simulink model "Porsche930Turbo_Model_V0"  (R2025b)
settings: Solver=ode3  StartTime=0.0  StopTime=1800  FixedStep=0.005  MaxStep=0.01  RelTol=1e-3
values from neighbouring files (symbols this model uses):
  a_front = (1 - CoG_front) * wb    (= 1.32912)    [Main.m]
  af = 1.77    [Main.m]
  bsfc = 395    [Main.m]
  cd = 0.39    [Main.m]
  crr = 0.015    [Main.m]
  distance_imola = s_track    [Main.m]
  eta_gb = 0.95    [Main.m]
  gear_numbers = [1, 2, 3, 4]    [Main.m]
  gear_ratios = [2.25, 1.30, 0.89, 0.625]    [Main.m]
  gear_shift_tbl = [1, 2, 3, 4]    [Main.m]
  grade_imola = grade_track    [Main.m]
  kt = 1.65    [Main.m]
  m_eq = mg + (J_wheels / rw^2) + (J_drivetrain * i_avg^2 / rw^2)    [Main.m]
  mg = mc + (mh * np) + mp_hybrid    (= 1492.5)    [Main.m]
  mu_road = 0.9    [Main.m]
  n_ice = 0:dn:nd    [Main.m]
  ne_em = 0:dn:nemax_em    [Main.m]
  nparallel = 2    [Main.m]
  nseries = 96    [Main.m]
  rho_fuel = 0.75    [Main.m]
  ro = 1.204    [Main.m]
  rt = 4.222    [Main.m]
  rw = (dw * 25.4 / 2 + wt * art / 100) * 1e-3    (= 0.31345)    [Main.m]
  t_ice = zeros(size(n_ice))    [Main.m]
  t_roma_san_basilio = [0 1 2 3 4 5 6 7 8 9 10 11 ... (522 elements, 522x1)]    [ECE_EUDC_Artemis_Bologna_Roma_WLTC_EE_bus.mat]
  tau_turbo = 0.6    [Main.m]
  te_em = zeros(size(ne_em))    [Main.m]
  te_em_peak = zeros(size(ne_em))    [Main.m]
  temax_em = 230    [Main.m]
  tmax_ice = 412    [Main.m]
  track_length = 4909    [Main.m]
  v_cutoff_bp = [0, 0.5, 1.4, 50]    [Main.m]
  v_cutoff_tbl = [0, 0,   1,   1 ]    [Main.m]
  v_ref_imola = v_track_ms    [Main.m]
  v_shift_bp = [0, 18, 33, 48]    [Main.m]
  v_shift_bp_EMODE = [0, 5, 22, 35]    [Main.m]
  vkm_roma_san_basilio = [28.8 30.9 32.4 34.2 35.3 35.6 34.8 33.8 32.2 30.5 29.1 27.9 ... (522 elements, 522x1)]    [ECE_EUDC_Artemis_Bologna_Roma_WLTC_EE_bus.mat]
  wb = 2.272    [Main.m]
undefined symbols (not defined in the file or in its folder): SoC_Per
libraries: simulink x58
(part 1 of 5)
settings Model: Creator=testi  LastModifiedBy=emanu
settings SolverCC: ConsecutiveZCsStepRelTol=1e-5  ZeroCrossAlgorithm=Adaptive
settings DebuggingCC: MergeDetectMultiDrivingBlocksExec=none  MaxConsecutiveZCsMsg=none  IgnoredZcDiagnostic=none
settings ModelReferenceCC: PropagateSignalLabelsOutOfModel=off

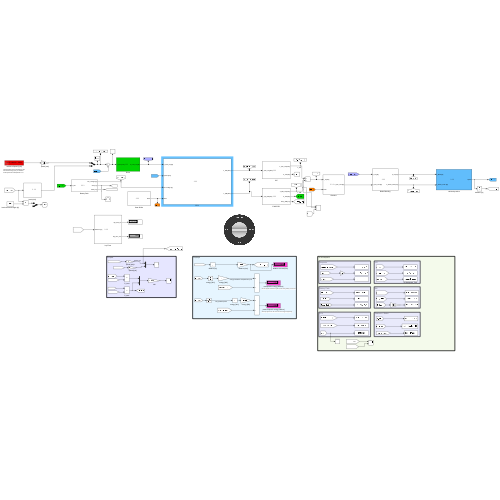
[thumbnail: Simulink's stored preview of the top-level diagram]
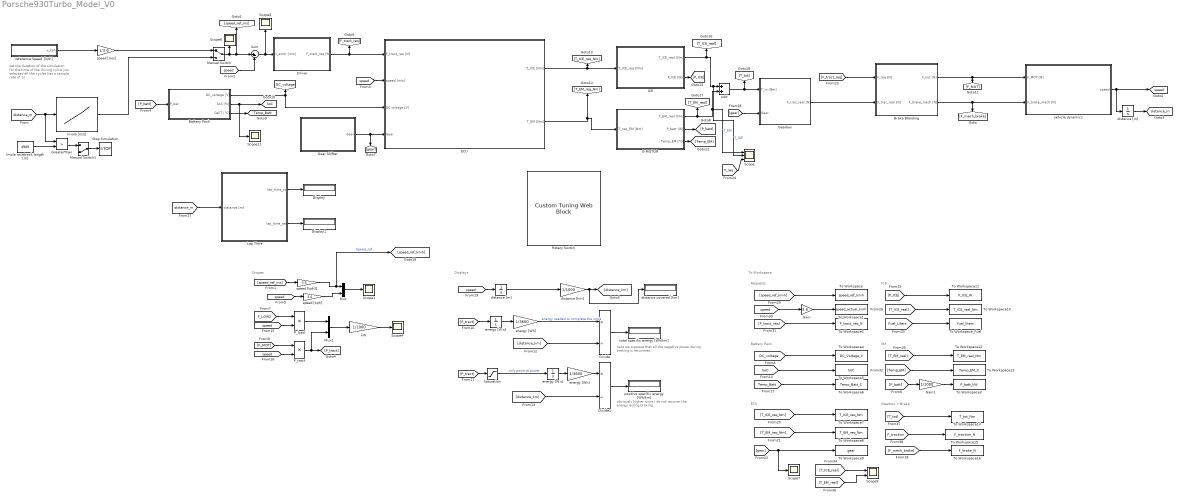
== system Porsche930Turbo_Model_V0 ==
  note: Gearbox + Brake
  note: EM
  note: ICE
  note: ECU
  note: Requests
  note: To Workspace
  note: set the duration of the simulation for the time of the driving cylce you selected
      | all the cycles has a sample rate of 1s
  note: Displays
  note: Scopes
  note: here we suppose that all the negative power during braking is recovered
  note: obviously higher since I do not recover the energy during braking
  note: Battery Pack
  Add : Sum
  Battery Pack : Subsystem
      mask Display: image('battery.jpg');
  Brake Blending : Subsystem
      mask Display: image('drumbrake.jpg');
  Display : Display
  Display1 : Display
  Divide : Product  Inputs=*/
  Divide1 : Product  Inputs=*/
  Driver : Subsystem
      mask Display: image('driver.webp');
  E-MOTOR : Subsystem
      mask Display: image('EMOTOR.jpg');
  ECU : Subsystem
      mask Display: image('ECU.webp');
  Gain : Gain  Gain=3.6
  Gain1 : Gain  Gain=1/1000
  Gear Shifter : Subsystem
      mask Display: image('Gearstick.jpeg');
  Gearbox : Subsystem
      mask Display: image('Gearbox.jpg');
  GreaterThan : RelationalOperator  Operator=>  OutDataTypeStr=boolean  RndMeth=Simplest  InputSameDT=off
  ICE : Subsystem
      mask Display: image('ICE.jpg');
  Imola [m/s] : Lookup_n-D  NumberOfTableDimensions=1  BreakpointsForDimension1=distance_imola  Table=v_ref_imola  InternalRulePriority=Speed  RndMeth=Simplest
      mask Display: image('imola.webp');
  Imola racetrack length [m] : Constant  Value=4909
  Lap TIme : Subsystem
      mask Display: image('clock.webp');
  Manual Switch : ManualSwitch
  Manual Switch1 : ManualSwitch  CurrentSetting=0
  Mux : Mux  Inputs=2
  Mux2 : Mux  Inputs=2
  P_load : Product
  P_tract : Product
  Rotary Switch : CustomTuningWebBlock  LabelPosition=Hide  ShowInitialText=on  Configuration="{\"components\":[{\"name\":\"RotarySwitchComponent\",\"settings\":{\"arcAngle\":270,\"arcAngleOffset\":180,\"handle\":{\"size\":[150,150],\"src\":\"data:image\\/svg+xml;base64,PHN2ZyBpZD0iTGF5ZXJfMSIgZGF0YS1uYW1lPSJMYXllciAxIiB4bWxucz0iaHR0cDovL3d3dy53My5vcmcvMjAwMC9zdmciIHhtbG5zOnhsaW5rPSJodHRwOi8vd3d3LnczLm9yZy8xOTk5L3hsaW5rIiB2aWV3Qm94PSIwIDAgMTIxIDEyMSI+PGRlZnM+PHN0eWxlPi5jbHMtMXtmaWxsOnVybCgjbGluZWFyLWdyYWRpZW50KTt9LmNscy0yLC5jbHMtM3tmaWxsOiNkMWQxZDE7fS5jbHMtM3tzdHJva2U6I2I3YjdiNztzdHJva2UtbWl0ZXJsaW1pdDoxMDtzdHJva2Utd2lkdGg6MC4yNXB4O30uY2xzLTR7ZmlsbDojZjMwMDAwO30uY2xzLTV7ZmlsbDojZjIxNzY3O308L3N0eWxlPjxsaW5lYXJHcmFkaWVudCBpZD0ibGluZWFyLWdyYWRpZW50IiB4MT0iNjAuNSIgeTE9IjEyMC41IiB4Mj0iNjAuNSIgeTI9IjAuNSIgZ3JhZGllbnRVbml0cz0idXNlclNwYWNlT25Vc2UiPjxzdG9wIG9mZnNldD0iMCIgc3RvcC1jb2xvcj0iI2QxZDFkMSIvPjxzdG9wIG9mZnNldD0iMC4xIiBzdG9wLWNvbG9yPSIjY2VjZWNlIi8+PHN0b3Agb2Zmc2V0PSIwLjE5IiBzdG9wLWNvbG9yPSIjYzNjM2MzIi8+PHN0b3Agb2Zmc2V0PSIwLjI4IiBzdG9wLWNvbG9yPSIjYjFiMWIxIi8+PHN0b3Agb2Zmc2V0PSIwLjM2IiBzdG9wLWNvbG9yPSIjOTg5ODk4Ii8+PHN0b3Agb2Zmc2V0PSIwLjQ0IiBzdG9wLWNvbG9yPSIjNzg3ODc4Ii8+PHN0b3Agb2Zmc2V0PSIwLjQ2IiBzdG9wLWNvbG9yPSIjNmI2YjZiIi8+PHN0b3Agb2Zmc2V0PSIwLjU0IiBzdG9wLWNvbG9yPSIjNmI2YjZiIi8+PHN0b3Agb2Zmc2V0PSIwLjU2IiBzdG9wLWNvbG9yPSIjNzY3Njc2Ii8+PHN0b3Agb2Zmc2V0PSIwLjY0IiBzdG9wLWNvbG9yPSIjOTc5Nzk3Ii8+PHN0b3Agb2Zmc2V0PSIwLjcyIiBzdG9wLWNvbG9yPSIjYjBiMGIwIi8+PHN0b3Agb2Zmc2V0PSIwLjgxIiBzdG9wLWNvbG9yPSIjYzNjM2MzIi8+PHN0b3Agb2Zmc2V0PSIwLjkiIHN0b3AtY29sb3I9IiNjZGNkY2QiLz48c3RvcCBvZmZzZXQ9IjEiIHN0b3AtY29sb3I9IiNkMWQxZDEiLz48L2xpbmVhckdyYWRpZW50PjwvZGVmcz48Y2lyY2xlIGNsYXNzPSJjbHMtMSIgY3g9IjYwLjUiIGN5PSI2MC41IiByPSI2MCIvPjxwYXRoIGNsYXNzPSJjbHMtMiIgZD0iTTYwLjUsMUE1OS41LDU5LjUsMCwxLDEsMSw2MC41LDU5LjU3LDU5LjU3LDAsMCwxLDYwLjUsMW0wLTFBNjAuNSw2MC41LDAsMSwwLDEyMSw2MC41LDYwLjUsNjAuNSwwLDAsMCw2MC41LDBaIi8+PHJlY3QgY2xhc3M9ImNscy0zIiB4PSIwLjUiIHk9IjUxLjUiIHdpZHRoPSIxMjAiIGhlaWdodD0iMTgiIHJ4PSIzLjA0Ii8+PHJlY3QgY2xhc3M9ImNscy00IiB4PSI1Ljc1IiB5PSI1OC43NSIgd2lkdGg9IjE2IiBoZWlnaHQ9IjMiLz48cGF0aCBjbGFzcz0iY2xzLTUiIGQ9Ik0yMS4yNSw1OS4yNXYyaC0xNXYtMmgxNW0xLTFoLTE3djRoMTd2LTRaIi8+PC9zdmc+\"},\"handleOffset\":[0,0],\"handleOrientation\":180,\"handlePosition\":[0,0,1,1],\"handleSize\":{\"height\":0.5,\"width\":0.5},\"labelRadius\":0.4,\"position\":[0,0,1,1],\"states\":[{\"Label\":{\"color\":[0,0,0,1],\"icon\":{\"size\":[0,0],\"src\":[],\"srcOrientation\":\"Right\"},\"iconOffset\":0,\"iconPlacement\":\"left\",\"opacity\":1,\"position\":[0.7345552884615385,0.6796274038461538],\"show\":true,\"text\":{\"content\":\"ICE\",\"font\":\"Helvetica\"}},\"Value\":1},{\"Label\":{\"color\":[0,0,0,1],\"icon\":{\"size\":[0,0],\"src\":[],\"srcOrientation\":\"Right\"},\"iconOffset\":0,\"iconPlacement\":\"left\",\"opacity\":1,\"position\":[0.35757211538461536,0.7603966346153846],\"show\":true,\"text\":{\"content\":\"ELECTRIC\",\"font\":\"Helvetica\"}},\"Value\":2},{\"Label\":{\"color\":[0,0,0,1],\"icon\":{\"size\":[0,0],\"src\":[],\"srcOrientation\":\"Right\"},\"iconOffset\":0,\"iconPlacement\":\"left\",\"opacity\":1,\"position\":[0.09603365384615385,0.46033653846153844],\"show\":true,\"text\":{\"content\":\"HYBRID\",\"font\":\"Helvetica\"}},\"Value\":3},{\"Label\":{\"color\":[0,0,0,1],\"icon\":{\"size\":[0,0],\"src\":[],\"srcOrientation\":\"Right\"},\"iconOffset\":0,\"iconPlacement\":\"left\",\"opacity\":1,\"position\":[0.36532451923076925,0.1180889423076923],\"show\":true,\"text\":{\"content\":\"RACE\",\"font\":\"Helvetica\"}},\"Value\":4}],\"tickRadius\":0.32}},{\"name\":\"BackgroundImageComponent\",\"settings\":{\"image\":{\"size\":[155,150],\"src\":\"data:image\\/svg+xml;base64,PD94bWwgdmVyc2lvbj0iMS4wIiBlbmNvZGluZz0idXRmLTgiPz4NCjwhLS0gR2VuZXJhdG9yOiBBZG9iZSBJbGx1c3RyYXRvciAyNS4wLjAsIFNWRyBFeHBvcnQgUGx1Zy1JbiAuIFNWRyBWZXJzaW9uOiA2LjAwIEJ1aWxkIDApICAtLT4NCjxzdmcgdmVyc2lvbj0iMS4xIg0KCSBpZD0iTGF5ZXJfMl8xXyIgeG1sbnM6Y2M9Imh0dHA6Ly9jcmVhdGl2ZWNvbW1vbnMub3JnL25zIyIgeG1sbnM6ZGM9Imh0dHA6Ly9wdXJsLm9yZy9kYy9lbGVtZW50cy8xLjEvIiB4bWxuczppbmtzY2FwZT0iaHR0cDovL3d3dy5pbmtzY2FwZS5vcmcv ...(+4184 chars)\",\"srcOrientation\":\"Right\"},\"position\":[0,0,1,1],\"scaleMode\":\"0\"}},{\"name\":\"ForegroundImageComponent\",\"settings\":{\"image\":{\"size\":[0,0],\"src\":\"default\",\"srcOrientation\":[]},\"isForeground\":1,\"position\":[0,0,1,1],\"scaleMode\":\"0\"}}],\"derived\":{\"blockParameters\":{\"ForegroundColor\":[0.9176470588235294,0.9176470588235294,0.9176470588235294],\"SelectedStateIndex\":0,\"States\":[{\"Label\":{\"color\":[0,0,0,1],\"icon\":{\"size\":[0,0],\"src\":[],\"srcOrientation\":\"Right\"},\"iconOffset\":0,\"iconPlacement\":\"left\",\"opacity\":1,\"position\":[0.7345552884615385,0.6796274038461538],\"show\":true,\"text\":{\"content\":\"ICE\",\"font\":\"Helvetica\"}},\"Value\":1},{\"Label\":{\"color\":[0,0,0,1],\"icon\":{\"size\":[0,0],\"src\":[],\"srcOrientation\":\"Right\"},\"iconOffset\":0,\"iconPlacement\":\"left\",\"opacity\":1,\"position\":[0.35757211538461536,0.7603966346153846],\"show\":true,\"text\":{\"content\":\"ELECTRIC\",\"font\":\"Helvetica\"}},\"Value\":2},{\"Label\":{\"color\":[0,0,0,1],\"icon\":{\"size\":[0,0],\"src\":[],\"srcOrientation\":\"Right\"},\"iconOffset\":0,\"iconPlacement\":\"left\",\"opacity\":1,\"position\":[0.09603365384615385,0.46033653846153844],\"show\":true,\"text\":{\"content\":\"HYBRID\",\"font\":\"Helvetica\"}},\"Value\":3},{\"Label\":{\"color\":[0,0,0,1],\"icon\":{\"size\":[0,0],\"src\":[],\"srcOrientation\":\"Right\"},\"iconOffset\":0,\"iconPlacement\":\"left\",\"opacity\":1,\"position\":[0.36532451923076925,0.1180889423076923],\"show\":true,\"text\":{\"content\":\"RACE\",\"font\":\"Helvetica\"}},\"Value\":4}],\"StatesJSON\":[{\"Label\":\"ICE\",\"Value\":1},{\"Label\":\"ELECTRIC\",\"Value\":2},{\"Label\":\"HYBRID\",\"Value\":3},{\"Label\":\"RACE\",\"Value\":4}],\"enumDataType\":\"\",\"fixedAspectRatio\":\"on\",\"useEnumDataType\":false}},\"settings\":{\"BindingType\":\"param\",\"backgroundColor\":[0,0,255,\"1\"],\"backgroundOffset\":1,\"fixedAspectRatio\":\"on\",\"image\":{\"size\":[150,150],\"src\":\"data:image\\/svg+xml;base64,PD94bWwgdmVyc2lvbj0iMS4wIiBlbmNvZGluZz0iVVRGLTgiIHN0YW5kYWxvbmU9Im5vIj8+CjwhLS0gR2VuZXJhdG9yOiBBZG9iZSBJbGx1c3RyYXRvciAxOS4yLjEsIFNWRyBFeHBvcnQgUGx1Zy1JbiAuIFNWRyBWZXJzaW9uOiA2LjAwIEJ1aWxkIDApICAtLT4KCjxzdmcKICAgeG1sbnM6ZGM9Imh0dHA6Ly9wdXJsLm9yZy9kYy9lbGVtZW50cy8xLjEvIgogICB4bWxuczpjYz0iaHR0cDovL2NyZWF0aXZlY29tbW9ucy5vcmcvbnMjIgogICB4bWxuczpyZGY9Imh0dHA6Ly93d3cudzMub3JnLzE5OTkvMDIvMjItcmRmLXN5bnRh ...(+9660 chars)\"},\"showBackgroundColor\":false,\"variant\":\"rotarySwitch\",\"version\":\"R2023a\"},\"type\":\"RotarySwitch\"}"  CustomBackgroundColor="{\"color\":[0,0,0],\"show\":true}"
  Saturation : Saturate  UpperLimit=inf  LowerLimit=0
  Scope : Scope  NumInputPorts=3
      settings: ActiveDisplayYMinimum=-46.9478660870644  ActiveDisplayYMaximum=422.53079478357967  DataLoggingVariableName=ScopeData11
  Scope{1,4..7,11} (6 alike) : Scope
      Scope1 settings: ActiveDisplayYMinimum=-21.249999999999996  ActiveDisplayYMaximum=191.25  DataLoggingVariableName=ScopeData18
      Scope11 settings: ActiveDisplayYMinimum=0.17583888024091721  ActiveDisplayYMaximum=0.417415089905262  DataLoggingVariableName=ScopeData37
      Scope4 settings: DataLoggingVariableName=ScopeData23
      Scope5 settings: ActiveDisplayYMinimum=-1  ActiveDisplayYMaximum=1  DataLoggingVariableName=ScopeData21
      Scope6 settings: ActiveDisplayYMinimum=-2.2361111111111112  ActiveDisplayYMaximum=20.125000000000004  DataLoggingVariableName=ScopeData22
      Scope7 settings: ActiveDisplayYMinimum=-1  ActiveDisplayYMaximum=1  DataLoggingVariableName=ScopeData29
  Scope9 : Scope  NumInputPorts=2
      settings: ActiveDisplayYMinimum=-51.4997582842605  ActiveDisplayYMaximum=463.49782455834463  DataLoggingVariableName=ScopeData31
  Stop Simulation : Stop
  Sum : Sum  Inputs=|+-
  To Workspace : ToWorkspace  VariableName=speed_ref_kmh  SampleTime=-1
  To Workspace1 : ToWorkspace  VariableName=speed_actual_kmh  SampleTime=-1
  To Workspace10 : ToWorkspace  VariableName=T_ICE_real_Nm  SampleTime=-1
  To Workspace11 : ToWorkspace  VariableName=P_ICE_W  SampleTime=-1
  To Workspace12 : ToWorkspace  VariableName=T_EM_real_Nm  SampleTime=-1
  To Workspace13 : ToWorkspace  VariableName=Temp_EM_C  SampleTime=-1
  To Workspace14 : ToWorkspace  VariableName=T_tot_Nm  SampleTime=-1
  To Workspace15 : ToWorkspace  VariableName=F_traction_N  SampleTime=-1
  To Workspace16 : ToWorkspace  VariableName=F_brake_N  SampleTime=-1
  To Workspace2 : ToWorkspace  VariableName=F_tract_req_N  SampleTime=-1
  To Workspace3 : ToWorkspace  VariableName=P_batt_kW  SampleTime=-1
  To Workspace4 : ToWorkspace  VariableName=DC_Voltage_V  SampleTime=-1
  To Workspace5 : ToWorkspace  VariableName=SoC  SampleTime=-1
  To Workspace6 : ToWorkspace  VariableName=Temp_Batt_C  SampleTime=-1
  To Workspace7 : ToWorkspace  VariableName=T_ICE_req_Nm  SampleTime=-1
  To Workspace8 : ToWorkspace  VariableName=T_EM_req_Nm  SampleTime=-1
  To Workspace9 : ToWorkspace  VariableName=gear  SampleTime=-1
  To Workspace_Fuel : ToWorkspace  VariableName=fuel_liters  SampleTime=-1
  distance [km] : Gain  Gain=1/1000
  distance [m] : Integrator
  "distance [m] " : Integrator
  distance covered [km] : Display
  energy [W.s] : Integrator
  "energy [W.s] " : Integrator
  energy [Wh] : Gain  Gain=1/3600
  "energy [Wh] " : Gain  Gain=1/3600
  kW : Gain  Gain=1/1000
  positive specific energy [Wh/km] : Display
  reference Speed  [kph] : Subsystem  mask{slct=WLTC class3b - 1800s}
      mask prompts: slct "Select Cycle"
      mask help: by mtb
      mask init:
      | load('ECE_EUDC_Artemis_Bologna_Roma_WLTC_EE_bus.mat')
      mask TypeOptions slct: ECE15 - 195s | EUDC - 400s | Art. Urban - 994s | Art. Rural - 1083s | Art. Motorway - 1068s | Roma S.Basilio - 522s | BO Viali slow - 1321s | BO Viali quick - 1215s | WLTC city - 1022s | WLTC class1 - 1612s | WLTC class2 - 1800s | WLTC class3a - 1800s | WLTC class3b - 1800s | Bus line BO 27A - 3246s | Bus line BO 27B - 3058s | Bus line BO 33 - 1850s | EE Bike Cycle - 1201s | 130kph
      mask DialogControl DescGroupVar Prompt: LEMAD Speed Cycle
      mask DialogControl DescTextVar Prompt: Function that outputs the speed reference in Km/h for the desired cycle
      mask Display:
      | switch slct
      |     case 1
      |         fprintf('ECE15 - 195s');
      |     case 2
      |         fprintf('EUDC - 400s');
      |     case 3
      |         fprintf('Art. Urban - 994s');
      |     case 4
      |         fprintf('Art. Rural - 1083s');
      |     case 5
      |         fprintf('Art. Motorway - 1068s');
      |     case 6
      |         fprintf('Roma S.Basilio - 522s');
      |     case 7
      |         fprintf('BO Viali slow - 1321s');
      |     case 8
      |         fprintf('BO Viali quick - 1215s');
      |     case 9
      |         fprintf('WLTC city - 1022s');
      |     case 10
      |         fprintf('WLTC class1 - 1612s');
      |     case 11
      |         fprintf('WLTC class2 - 1800s');
      |     case 12
      |         fprintf('WLTC class3a - 1800s');
      |     case 13
      |         fprintf('WLTC class3b - 1800s');
      |     case 14
      |         fprintf('Bus line BO 27A - 3246s');
      |     case 15
      |         fprintf('Bus line BO 27A - 3058s');
      |     case 16
      |         fprintf('Bus line BO 33 - 1850s');
      |     case 17
      |         fprintf('EE Bike Cycle - 1201s');
      |     case 18
      |         fprintf('130kph');
      | end
  speed [kph] : Gain  Gain=3.6
  speed [kph]1 : Gain  Gain=3.6
  speed [m/s] : Gain  Gain=1/3.6
  total specific energy [Wh/km] : Display
  vehicle dynamics : Subsystem
      mask Display: image('930_turbo_050.webp');
  tag scope: DC_voltage=global, SoC=global, Temp_Batt=global, distance_m=global, speed=global
  wires:
  Sum/1 -> Driver/1(v_error [m/s]), Scope5/1
  Driver/1(F_tract_req [N]) -> [F_tract_req], ECU/1(F_tract_req [N])
  Battery Pack/1(DC_voltage [V]) -> ECU/3(DC voltage [V]), [DC_voltage]
  ECU/1(T_ICE [Nm]) -> ICE/1(T_ICE_req [Nm]), [T_ICE_req_Nm]
  ICE/1(T_ICE_real [Nm]) -> [T_ICE_real], Scope/2, Add/1  "T_ICE"
  [P_tract] -> energy [W.s]/1
  Mux2/1 -> kW/1
  [distance_km] -> Divide1/2
  Saturation/1 -> "energy [W.s] "/1  "only positive power"
  "energy [Wh] "/1 -> Divide1/1
  kW/1 -> Scope4/1
  Divide1/1 -> positive specific energy [Wh/km]/1
  P_tract/1 -> Mux2/2, [P_tract]
  "energy [W.s] "/1 -> "energy [Wh] "/1
  [speed] -> speed [kph]/1
  Mux/1 -> Scope1/1
  [F_LOAD] -> P_load/1
  [speed] -> P_tract/2
  energy [Wh]/1 -> Divide/1  "energy needed to complete the cycle"
  [distance_km] -> Divide/2
  [P_tract] -> Saturation/1
  [speed] -> distance [m]/1
  [speed] -> P_load/2
  [speed_ref_ms] -> speed [kph]1/1
  distance [km]/1 -> distance covered [km]/1, [distance_km]
  speed [kph]/1 -> Mux/2
  Divide/1 -> total specific energy [Wh/km]/1
  [F_MOT] -> P_tract/1
  energy [W.s]/1 -> energy [Wh]/1
  P_load/1 -> Mux2/1
  distance [m]/1 -> distance [km]/1
  [F_tract_req] -> Brake Blending/1(F_req [N])
  Brake Blending/1(F_out [N]) -> [F_MOT], vehicle dynamics/1(F_MOT [N])
  Brake Blending/2(F_brake_mech [N]) -> vehicle dynamics/2(F_brake_mech [N]), [F_mech_brake]
  [P_batt] -> Battery Pack/1(P_bat)
  vehicle dynamics/1(speed) -> "distance [m] "/1, [speed]
  "distance [m] "/1 -> [distance_m]
  [distance_m] -> GreaterThan/1, Imola [m/s]/1
  Imola [m/s]/1 -> Manual Switch/2
  speed [m/s]/1 -> Manual Switch/1
  Manual Switch/1 -> [speed_ref_ms], Sum/1, Scope6/1
  Add/1 -> [T_tot], Gearbox/1(T_in [Nm])
  Imola racetrack length [m]/1 -> GreaterThan/2
  [gear] -> Gearbox/2(Gear)
  Gearbox/1(F_trac_real [N]) -> Brake Blending/2(F_trac_real [N])
  E-MOTOR/2(P_batt [W]) -> [P_batt]
  Battery Pack/3(CellT [°C]) -> [Temp_Batt]
  E-MOTOR/1(T_EM_real [Nm]) -> [T_EM_real], Add/2, Scope/1  "T_EM"
  Battery Pack/2(SoC [%]) -> Scope11/1, [SoC]
  [distance_m] -> Lap TIme/1(distance [m])
  Lap TIme/1(lap_time_str) -> Display/1
  Lap TIme/2(lap_time_sec) -> Display1/1
  reference Speed  [kph]/1(v_kph) -> speed [m/s]/1
  GreaterThan/1 -> Manual Switch1/1
  Manual Switch1/1 -> Stop Simulation/1
  E-MOTOR/3(Temp_EM [°C]) -> [Temp_EM]
  [speed] -> Gain/1
  [speed_ref_kmh] -> To Workspace/1
  Gain/1 -> To Workspace1/1
  [F_tract_req] -> To Workspace2/1
  [SoC] -> To Workspace5/1
  [DC_voltage] -> To Workspace4/1
  [Temp_Batt] -> To Workspace6/1
  [speed] -> ECU/2(speed [m/s])
  [speed] -> Sum/2
  ECU/2(T_EM [Nm]) -> [T_EM_req_Nm], E-MOTOR/1(T_req_EM [Nm])
  [T_ICE_req_Nm] -> To Workspace7/1
  [T_EM_req_Nm] -> To Workspace8/1
  [gear] -> Scope7/1, To Workspace9/1
  ICE/2(P_ICE [W]) -> [P_ICE]
  [Fuel_Liters] -> To Workspace_Fuel/1
  [T_ICE_real] -> To Workspace10/1
  [P_ICE] -> To Workspace11/1
  [T_ICE_real] -> Scope9/1
  [P_batt] -> Gain1/1
  Gain1/1 -> To Workspace3/1
  [Temp_EM] -> To Workspace13/1
  [T_EM_real] -> To Workspace12/1
  [T_EM_real] -> Scope9/2
  [T_tot] -> To Workspace14/1
  [F_traction] -> To Workspace15/1
  Gear Shifter/1(Gear) -> ECU/4(Gear), [gear]
  [F_mech_brake] -> To Workspace16/1
  speed [kph]1/1 -> [speed_ref_kmh], Mux/1  "Speed_ref"
  [T_req] -> Scope/3

== system Porsche930Turbo_Model_V0/Battery Pack ==
  P_bat : Inport
  " " : Product  Inputs=*/
  Constant : Constant  Value=25
  Constant1 : Constant  Value=nparallel
  Constant2 : Constant  Value=nseries
  Data Type Conversion : DataTypeConversion  SaturateOnIntegerOverflow=off  RndMeth=Floor
  Gain2 : Gain  Gain=1/100
  Memory : Memory  InitialCondition=345.2
  P_tract1 : Product  Inputs=3
  Scope : Scope
      settings: ActiveDisplayYMinimum=271.806844329834  ActiveDisplayYMaximum=353.35479507446286  DataLoggingVariableName=ScopeData36
  Scope2 : Scope  NumInputPorts=4
      settings: Title=BATTERY VOLTAGE  ActiveDisplayYMinimum=338.44709014892578  ActiveDisplayYMaximum=434.32286834716797  DataLoggingSaveFormat=Array
  Subsystem : Subsystem  mask{seriesNumber=96, parallelNumber=2, InitialSOC=SoC_Per, InitialSOH=100.0, BattEff=98.0, CellType=MOLICEL	21700	P42A	4.2 [Ah], ThermalModelType=1D With Plastic, ThermReff=off, TRoom=20.300, R1Therml=2.4, R2Therml=8e-4, R3Therml=9, C1Thermal=62, C2Thermal=4.5}
      mask prompts: seriesNumber "Series Moduels Number [/]"; parallelNumber "Parallel Moduels Number [/]"; InitialSOC "Initial SoC value [%]"; InitialSOH "Initial SoH value [%]"; BattEff "Battery Efficency [%]  (Beta)"; CellType "Cell Type"; ThermalModelType "Thermal Model Type"; ThermReff "Internal Reference"; TRoom "Room Temperautre [°C]"; R1Therml "Core Resistence (R1)  [K/W]"; R2Therml "Can Resistence (R2)  [K/W]"; R3Therml "External Resistence (R3)  [K/W]"; C1Thermal "Core Capacity (C1) [J/K]"; C2Thermal "Can Capacity (C2) [J/K]"
      mask init:
      | if ~exist('batCoeffStudent', 'var')
      |     load('batCoeffStudent.mat')
      | end
      | 
      | switch CellType
      |     case 1 %'IFR18650 EC'
      |         CellNum = 3;
      |     case 2 %'NCR18650 B'
      |         CellNum = 2;
      |     case 3 % NCR18650 GA
      |         CellNum = 4;
      |     case 4 %'INR18650 S'
      |         CellNum = 10;
      |     case 5 %'INR21700 E'
      |         CellNum = 11;
      |     case 6 %'INR21700 S'
      |         CellNum = 12;
      |     case 7 %'INR18650 VTC6'
      |         CellNum = 13;
      |     case 8 %'INR21700 VTC6A'
      |         CellNum = 14;
      |     case 9 % 'INR21700 M50T'
      |         CellNum = 6;
      |     case 10 % 'INR21700 M50T'
      |         CellNum = 5;
      |     case 11 % 'INR21700 P42A'
      |         CellNum = 7;
      |     case 12 % 'INR21700 K42'
      |         CellNum = 8;
      |     case 13 % 'INR21700 K42X'
      |         CellNum = 9;
      | end
      | j = 3;
      | batFormat = batCoeff{CellNum, j};j = j + 1;
      | cellCapacity = batCoeff{CellNum, j};
      | j = 6;
      | voltLim = batCoeff{CellNum, j};j = j + 1;
      | currLim = batCoeff{CellNum, j};
      | j = 8;
      | voc = batCoeff{CellNum, j};j = j + 1;
      | dvoc = batCoeff{CellNum, j};j = j + 1;
      | Cp = batCoeff{CellNum, j};j = j + 1;
      | R0 = batCoeff{CellNum, j};j = j + 1;
      | R0T = batCoeff{CellNum, j};j = j + 1;
      | R0SOH = batCoeff{CellNum, j};j = j + 1;
      | R1 = batCoeff{CellNum, j};j = j + 1;
      | R1T = batCoeff{CellNum, j};j = j + 1;
      | tau1 = batCoeff{CellNum, j};
      mask TypeOptions CellType: OCELL	18650	EC	1.5 [Ah] | PANASONIC	18650	B	3.2 [Ah] | PANASONIC	18650	GA	3.35 [Ah] | SAMSUNG	18650 	35E	3.35 [Ah] | SAMSUNG	21700 	50E	4.9 [Ah] | SAMSUNG	21700 	50S	5 [Ah] | MURATA 	18650	VTC6	3.12 [Ah] | MURATA 	21700	VTC6A	4 [Ah] | LG	21700 	M50T	5 [Ah] | MOLICEL 	21700	M50A	5 [Ah] | MOLICEL	21700	P42A	4.2 [Ah] | KEEPPOWER	21700	K42	4.2 [Ah] | KEEPPOWER	21700	K42X	4.2 [Ah]
      mask TypeOptions ThermalModelType: Constant | 1D With Plastic | 1D No Plastic
      mask DialogControl Container13 Prompt: Pack Parameters
      mask DialogControl Container7 Prompt: Pack Configuration
      mask DialogControl Container14 Prompt: Thermal Parameters
      mask DialogControl Container6 Prompt: Room Temperature
      mask DialogControl Container15 Prompt: Thermal Parameters
      mask Display:
      | fprintf('Discrete Battery Model \n \n \n');
      | fprintf('V 0.3.2');
      | fprintf('\n\n\n %ds%dp %s \n%5.1f[Ah]', seriesNumber,parallelNumber,batFormat, cellCapacity*parallelNumber)
      | 
      | set_param(gcb,'MaskHideContents','off')
  Transfer Fcn1 : TransferFcn  Denominator=[0.01 1]
  parallel : Gain  Gain=1/nparallel
  DC_voltage [V] : Outport
  SoC [%] : Outport  Port=2
  CellT [°C] : Outport  Port=3
  wires:
  Memory/1 -> Transfer Fcn1/1, " "/2, Scope2/1, Scope/1  "battery voltage"
  Subsystem/4(PowrLoss(t) [W]) -> P_tract1/1
  Gain2/1 -> SoC [%]/1
  Constant1/1 -> P_tract1/2
  Subsystem/3(SOC [%]) -> Gain2/1, Scope2/3
  P_bat/1 -> " "/1
  Subsystem/1(vB [V]) -> Data Type Conversion/1  "real"
  " "/1 -> parallel/1  "battery current"
  P_tract1/1 -> Scope2/4
  Data Type Conversion/1 -> Memory/1
  parallel/1 -> Subsystem/1(iB [A])  "cell current"
  Constant/1 -> Subsystem/2(TAmb [°C])
  Subsystem/2(CellT [°C]) -> CellT [°C]/1, Scope2/2
  Constant2/1 -> P_tract1/3
  Transfer Fcn1/1 -> DC_voltage [V]/1

== system Porsche930Turbo_Model_V0/Brake Blending ==
  F_req [N] : Inport
  F_trac_real [N] : Inport  Port=2
  " " : Constant  Value=0
  Is_Braking : simulink/Logic and Bit Operations/Compare To Constant  relop=<=  const=0  OutDataTypeStr=boolean
  Sub_Mech : Sum  Inputs=+-
  Switch_Brake_Mech : Switch  Criteria=u2 > Threshold  Threshold=0.5  SaturateOnIntegerOverflow=off  InputSameDT=off
  F_out [N] : Outport
  F_brake_mech [N] : Outport  Port=2
  wires:
  Is_Braking/1 -> Switch_Brake_Mech/2
  Sub_Mech/1 -> Switch_Brake_Mech/1
  " "/1 -> Switch_Brake_Mech/3
  Switch_Brake_Mech/1 -> F_brake_mech [N]/1
  F_req [N]/1 -> Is_Braking/1, Sub_Mech/1
  F_trac_real [N]/1 -> F_out [N]/1, Sub_Mech/2

== system Porsche930Turbo_Model_V0/Driver ==
  v_error [m/s] : Inport
  Add : Sum
  Constant : Constant  Value=-mu_road*9.81*mg
  Constant1 : Constant  Value=mu_road * mg * 9.81 * (a_front / wb)
  Gain : Gain  Gain=500
  Integrator Limited : Integrator  LimitOutput=on  LowerSaturationLimit=0
  KI : Gain  Gain=10000
  KP : Gain  Gain=7000
  Saturation Dynamic : simulink/Discontinuities/Saturation Dynamic  OutMin=[]  OutMax=[]  OutDataTypeStr=Inherit: Same as second input  OutDataType=fixdt(1, 16)  OutScaling=2^-10  DoSatur=off
  Subtract : Sum  Inputs=-+
  Sum : Sum  Inputs=|+-
  F_tract_req [N] : Outport
  wires:
  v_error [m/s]/1 -> KI/1, KP/1
  KP/1 -> Add/1
  Sum/1 -> Integrator Limited/1
  Add/1 -> Subtract/2, Saturation Dynamic/2
  Subtract/1 -> Gain/1
  Gain/1 -> [diff]
  KI/1 -> Sum/1
  [diff] -> Sum/2
  Constant/1 -> Saturation Dynamic/3
  Constant1/1 -> Saturation Dynamic/1
  Saturation Dynamic/1 -> F_tract_req [N]/1, Subtract/1
  Integrator Limited/1 -> Add/2
